simulink library "bat_13S7P_detailed"  (R2025b)
settings: Solver=VariableStepAuto  StartTime=0.0  StopTime=10.0  RelTol=1e-3
undefined symbols (not defined in the file or in its folder): battery_builder_rtmsupport, gcbh
libraries: bat_13S7P_detailed_lib x14
settings Model: Creator=scb4  LastModifiedBy=scb4

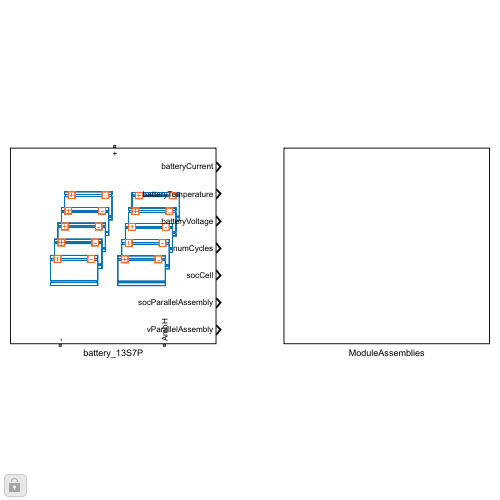
[thumbnail: Simulink's stored preview of the top-level diagram]
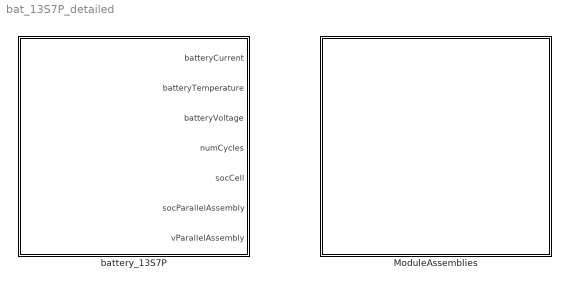
== system bat_13S7P_detailed ==
  ModuleAssemblies : Subsystem
  battery_13S7P : Subsystem  LoadFcn=battery_builder_rtmsupport('loadfcn',gcbh);
      settings: CopyFcn=battery_builder_rtmsupport('copyfcn',gcbh);  PreCopyFcn=battery_builder_rtmsupport('precopyfcn',gcbh);  PreDeleteFcn=battery_builder_rtmsupport('predeletefcn',gcbh);  PortSchema="{\"entries\":[{\"content\":{\"sides\":[{\"content\":{\"connectorIds\":[\"LConn1\"]},\"type\":\"ConnectorPlacement.EquallySpacedRectSide\",\"uuid\":\"c922c71b-bb80-4818-bdc8-e90d40dfbbb3\"},{\"content\":{\"connectorIds\":[\"RConn1\",\"RConn2\"],\"side\":\"RIGHT\"},\"type\":\"ConnectorPlacement.EquallySpacedRectSide\",\"uuid\":\"8cfcb0b4-3cbc-4068-a33f-0ddf2418c87b\"},{\"content\":{\"side\":\"TOP\"},\"type\":\"ConnectorPlacement.EquallySpacedRectSide\",\"uuid\":\"a3bda4bf-8d06-4bf0-ab5f-e835ee1e9452\"},{\"content\":{\"connectorIds\":[\"Out1\",\"Out2\",\"Out3\",\"Out4\",\"Out5\",\"Out6\",\"Out7\"],\"side\":\"BOTTOM\"},\"type\":\"ConnectorPlacement.EquallySpacedRectSide\",\"uuid\":\"4dc4e40d-eeb2-4e6c-ad84-aff3d30c3561\"}]},\"type\":\"ConnectorPlacement.EquallySpacedConnector\",\"uuid\":\"9bf5a596-b0f6-40a9-8ffe-ca0735a12662\"}],\"packageUris\":[\"http://schema.mathworks.com/mf0/Connector/R2020b\"],\"version\":\"1.0\"}"
      mask Display: image('$imagefile')

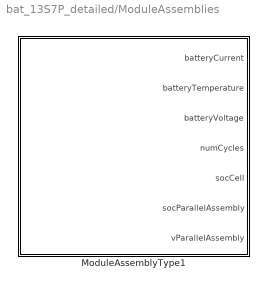
== system bat_13S7P_detailed/ModuleAssemblies ==
  ModuleAssemblyType1 : Subsystem  LoadFcn=battery_builder_rtmsupport('loadfcn',gcbh);
      settings: CopyFcn=battery_builder_rtmsupport('copyfcn',gcbh);  PreCopyFcn=battery_builder_rtmsupport('precopyfcn',gcbh);  PreDeleteFcn=battery_builder_rtmsupport('predeletefcn',gcbh);  PortSchema="{\"entries\":[{\"content\":{\"sides\":[{\"content\":{\"connectorIds\":[\"LConn1\"]},\"type\":\"ConnectorPlacement.EquallySpacedRectSide\",\"uuid\":\"c922c71b-bb80-4818-bdc8-e90d40dfbbb3\"},{\"content\":{\"connectorIds\":[\"RConn1\",\"RConn2\"],\"side\":\"RIGHT\"},\"type\":\"ConnectorPlacement.EquallySpacedRectSide\",\"uuid\":\"8cfcb0b4-3cbc-4068-a33f-0ddf2418c87b\"},{\"content\":{\"side\":\"TOP\"},\"type\":\"ConnectorPlacement.EquallySpacedRectSide\",\"uuid\":\"a3bda4bf-8d06-4bf0-ab5f-e835ee1e9452\"},{\"content\":{\"connectorIds\":[\"Out1\",\"Out2\",\"Out3\",\"Out4\",\"Out5\",\"Out6\",\"Out7\"],\"side\":\"BOTTOM\"},\"type\":\"ConnectorPlacement.EquallySpacedRectSide\",\"uuid\":\"a7aca7be-b7c9-453c-ab2d-6778c2fb4d01\"}]},\"type\":\"ConnectorPlacement.EquallySpacedConnector\",\"uuid\":\"9bf5a596-b0f6-40a9-8ffe-ca0735a12662\"}],\"packageUris\":[\"http://schema.mathworks.com/mf0/Connector/R2020b\"],\"version\":\"1.0\"}"
      mask Display: image('$imagefile')

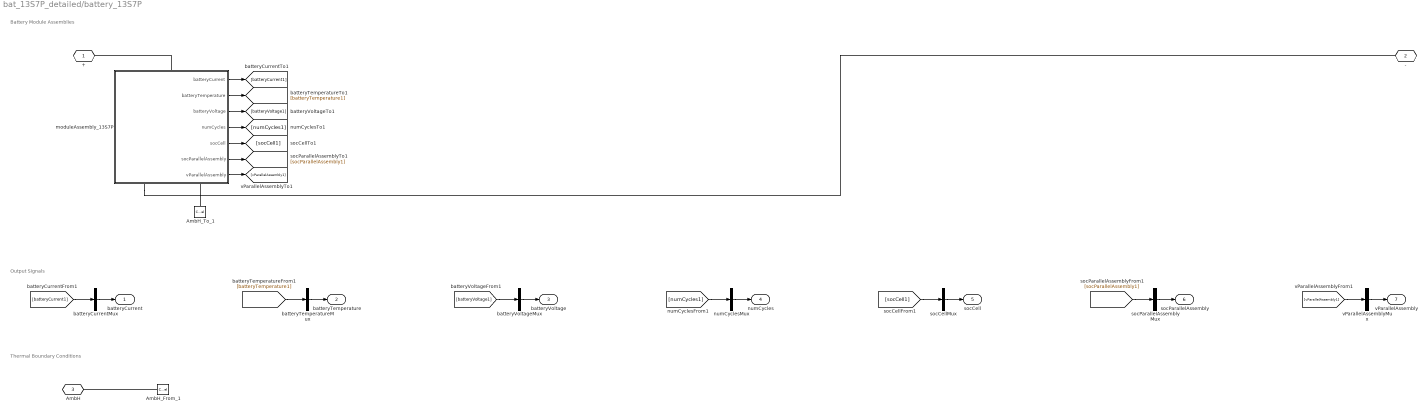
== system bat_13S7P_detailed/battery_13S7P ==
  note: Battery Module Assemblies
  note: Output Signals
  note: Thermal Boundary Conditions
  AmbH_From_1 : ConnectionLabel  Label=ambH_1
  AmbH_To_1 : ConnectionLabel  Label=ambH_1
  batteryCurrentMux : Mux  Inputs=1
  batteryTemperatureMux : Mux  Inputs=1
  batteryVoltageMux : Mux  Inputs=1
  moduleAssembly_13S7P : Subsystem  LoadFcn=battery_builder_rtmsupport('loadfcn',gcbh);
      settings: CopyFcn=battery_builder_rtmsupport('copyfcn',gcbh);  PreCopyFcn=battery_builder_rtmsupport('precopyfcn',gcbh);  PreDeleteFcn=battery_builder_rtmsupport('predeletefcn',gcbh);  PortSchema="{\"entries\":[{\"content\":{\"sides\":[{\"content\":{\"connectorIds\":[\"LConn1\"]},\"type\":\"ConnectorPlacement.EquallySpacedRectSide\",\"uuid\":\"c922c71b-bb80-4818-bdc8-e90d40dfbbb3\"},{\"content\":{\"connectorIds\":[\"RConn1\",\"RConn2\"],\"side\":\"RIGHT\"},\"type\":\"ConnectorPlacement.EquallySpacedRectSide\",\"uuid\":\"8cfcb0b4-3cbc-4068-a33f-0ddf2418c87b\"},{\"content\":{\"side\":\"TOP\"},\"type\":\"ConnectorPlacement.EquallySpacedRectSide\",\"uuid\":\"a3bda4bf-8d06-4bf0-ab5f-e835ee1e9452\"},{\"content\":{\"connectorIds\":[\"Out1\",\"Out2\",\"Out3\",\"Out4\",\"Out5\",\"Out6\",\"Out7\"],\"side\":\"BOTTOM\"},\"type\":\"ConnectorPlacement.EquallySpacedRectSide\",\"uuid\":\"a7aca7be-b7c9-453c-ab2d-6778c2fb4d01\"}]},\"type\":\"ConnectorPlacement.EquallySpacedConnector\",\"uuid\":\"9bf5a596-b0f6-40a9-8ffe-ca0735a12662\"}],\"packageUris\":[\"http://schema.mathworks.com/mf0/Connector/R2020b\"],\"version\":\"1.0\"}"
      mask Display: image('$imagefile')
  numCyclesMux : Mux  Inputs=1
  socCellMux : Mux  Inputs=1
  socParallelAssemblyMux : Mux  Inputs=1
  vParallelAssemblyMux : Mux  Inputs=1
  + : PMIOPort  Side=Left
  - : PMIOPort  Port=2  Side=Right
  AmbH : PMIOPort  Port=3  Side=Right  ConnectionType=Connection: foundation.thermal.thermal
  batteryCurrent : Outport
  batteryTemperature : Outport  Port=2
  batteryVoltage : Outport  Port=3
  numCycles : Outport  Port=4
  socCell : Outport  Port=5
  socParallelAssembly : Outport  Port=6
  vParallelAssembly : Outport  Port=7
  wires:
  moduleAssembly_13S7P/1(batteryCurrent) -> [batteryCurrent1]
  batteryCurrentMux/1 -> batteryCurrent/1
  [batteryCurrent1] -> batteryCurrentMux/1
  moduleAssembly_13S7P/2(batteryTemperature) -> [batteryTemperature1]
  batteryTemperatureMux/1 -> batteryTemperature/1
  [batteryTemperature1] -> batteryTemperatureMux/1
  moduleAssembly_13S7P/3(batteryVoltage) -> [batteryVoltage1]
  batteryVoltageMux/1 -> batteryVoltage/1
  [batteryVoltage1] -> batteryVoltageMux/1
  moduleAssembly_13S7P/4(numCycles) -> [numCycles1]
  numCyclesMux/1 -> numCycles/1
  [numCycles1] -> numCyclesMux/1
  moduleAssembly_13S7P/5(socCell) -> [socCell1]
  socCellMux/1 -> socCell/1
  [socCell1] -> socCellMux/1
  moduleAssembly_13S7P/6(socParallelAssembly) -> [socParallelAssembly1]
  socParallelAssemblyMux/1 -> socParallelAssembly/1
  [socParallelAssembly1] -> socParallelAssemblyMux/1
  moduleAssembly_13S7P/7(vParallelAssembly) -> [vParallelAssembly1]
  vParallelAssemblyMux/1 -> vParallelAssembly/1
  [vParallelAssembly1] -> vParallelAssemblyMux/1
  connections:
  moduleAssembly_13S7P/LConn1 -- +/RConn1
  moduleAssembly_13S7P/RConn1 -- -/RConn1
  AmbH_To_1/LConn1 -- moduleAssembly_13S7P/RConn2
  AmbH_From_1/LConn1 -- AmbH/RConn1

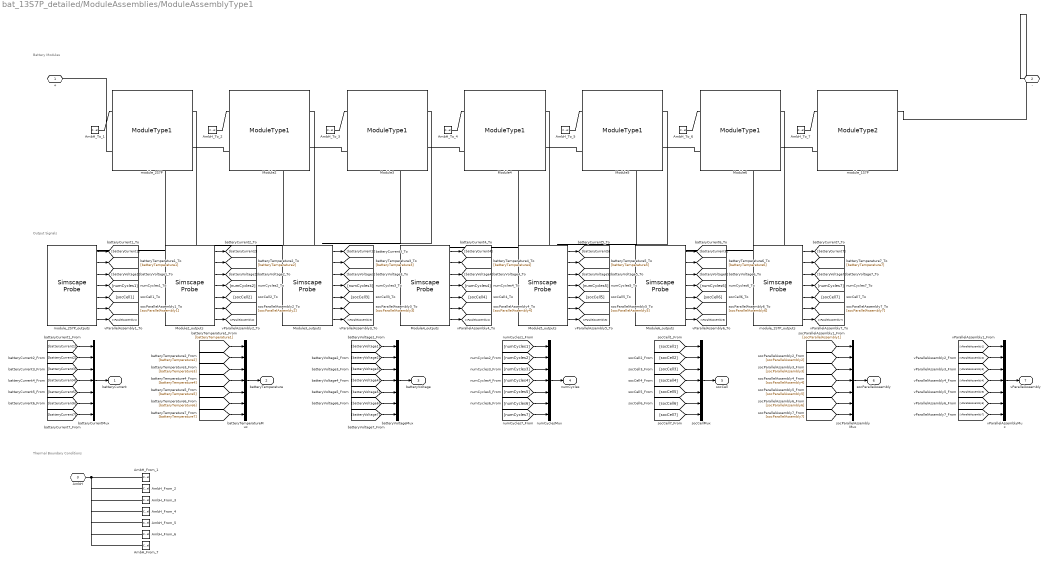
== system bat_13S7P_detailed/ModuleAssemblies/ModuleAssemblyType1 ==
  note: Battery Modules
  note: Output Signals
  note: Thermal Boundary Conditions
  AmbH_From_1 : ConnectionLabel  Label=ambH_1
  AmbH_From_2 : ConnectionLabel  Label=ambH_2
  AmbH_From_3 : ConnectionLabel  Label=ambH_3
  AmbH_From_4 : ConnectionLabel  Label=ambH_4
  AmbH_From_5 : ConnectionLabel  Label=ambH_5
  AmbH_From_6 : ConnectionLabel  Label=ambH_6
  AmbH_From_7 : ConnectionLabel  Label=ambH_7
  AmbH_To_1 : ConnectionLabel  Label=ambH_1
  AmbH_To_2 : ConnectionLabel  Label=ambH_2
  AmbH_To_3 : ConnectionLabel  Label=ambH_3
  AmbH_To_4 : ConnectionLabel  Label=ambH_4
  AmbH_To_5 : ConnectionLabel  Label=ambH_5
  AmbH_To_6 : ConnectionLabel  Label=ambH_6
  AmbH_To_7 : ConnectionLabel  Label=ambH_7
  Module{2..6} (5 alike) : bat_13S7P_detailed_lib/Modules/ModuleType1  BatteryCapacityCell=ModuleType1.BatteryCapacityCell A*hr  ExtrapolationMethodCell=simscape.enum.extrapolation.nearest  SOCBreakpointsCell=ModuleType1.SOCBreakpointsCell  TemperatureBreakpointsCell=ModuleType1.TemperatureBreakpointsCell K  OpenCircuitVoltageThermalCell=ModuleType1.OpenCircuitVoltageThermalCell V  VoltageRangeCell=ModuleType1.VoltageRangeCell V  ResistanceSOCBreakpointsCell=ModuleType1.ResistanceSOCBreakpointsCell  ResistanceTemperatureBreakpointsCell=ModuleType1.ResistanceTemperatureBreakpointsCell K  R0ThermalCell=ModuleType1.R0ThermalCell Ohm  R1ThermalCell=ModuleType1.R1ThermalCell Ohm  Tau1ThermalCell=ModuleType1.Tau1ThermalCell s  BatteryThermalMassCell=ModuleType1.BatteryThermalMassCell J/K  AmbientResistance=ModuleType1.AmbientResistance K/W  P=7  S=2  socCell_specify=off  socCell_priority=High  socCell=repmat(1, 14, 1)  socCell_nominal_specify=off  socCell_nominal_value=1  socCell_nominal_unit=1  batteryVoltage_specify=off  batteryVoltage_priority=None  batteryVoltage=repmat(0, 14, 1) V  batteryVoltage_nominal_specify=off  batteryVoltage_nominal_value=1  batteryVoltage_nominal_unit=V  batteryCurrent_specify=off  batteryCurrent_priority=None  batteryCurrent=repmat(0, 14, 1) A  batteryCurrent_nominal_specify=off  batteryCurrent_nominal_value=1  batteryCurrent_nominal_unit=A  numCycles_specify=off  numCycles_priority=High  numCycles=repmat(0, 14, 1)  numCycles_nominal_specify=off  numCycles_nominal_value=1  numCycles_nominal_unit=1  batteryTemperature_specify=off  batteryTemperature_priority=High  batteryTemperature=repmat(298.15, 14, 1) K  batteryTemperature_nominal_specify=off  batteryTemperature_nominal_value=1  batteryTemperature_nominal_unit=K  vParallelAssembly_specify=off  vParallelAssembly_priority=None  vParallelAssembly=repmat(0, 2, 1) V  vParallelAssembly_nominal_specify=off  vParallelAssembly_nominal_value=1  vParallelAssembly_nominal_unit=V  socParallelAssembly_specify=off  socParallelAssembly_priority=None  socParallelAssembly=repmat(1, 2, 1)  socParallelAssembly_nominal_specify=off  socParallelAssembly_nominal_value=1  socParallelAssembly_nominal_unit=1
      settings: InternalSimscapePortConfiguration="{\"Bottom\":[{\"id\":\"n\",\"label\":\"-\",\"type\":\"foundation.electrical.electrical\"},{\"id\":\"BottomExtClnt\",\"label\":\"CPB\",\"type\":\"foundation.thermal.thermal\"}],\"Left\":[{\"id\":\"AmbH\",\"label\":\"AmbH\",\"type\":\"foundation.thermal.thermal\"}],\"Right\":[],\"Top\":[{\"id\":\"p\",\"label\":\"+\",\"type\":\"foundation.electrical.electrical\"}]}"
  Module2_outputs : SimscapeProbe  BoundBlock=4  Variables="{\"batteryCurrent\":{\"Probing\":\"ON\"},\"batteryTemperature\":{\"Probing\":\"ON\"},\"batteryVoltage\":{\"Probing\":\"ON\"},\"numCycles\":{\"Probing\":\"ON\"},\"socCell\":{\"Probing\":\"ON\"},\"socParallelAssembly\":{\"Probing\":\"ON\"},\"vParallelAssembly\":{\"Probing\":\"ON\"}}"
  Module3_outputs : SimscapeProbe  BoundBlock=5  Variables="{\"batteryCurrent\":{\"Probing\":\"ON\"},\"batteryTemperature\":{\"Probing\":\"ON\"},\"batteryVoltage\":{\"Probing\":\"ON\"},\"numCycles\":{\"Probing\":\"ON\"},\"socCell\":{\"Probing\":\"ON\"},\"socParallelAssembly\":{\"Probing\":\"ON\"},\"vParallelAssembly\":{\"Probing\":\"ON\"}}"
  Module4_outputs : SimscapeProbe  BoundBlock=6  Variables="{\"batteryCurrent\":{\"Probing\":\"ON\"},\"batteryTemperature\":{\"Probing\":\"ON\"},\"batteryVoltage\":{\"Probing\":\"ON\"},\"numCycles\":{\"Probing\":\"ON\"},\"socCell\":{\"Probing\":\"ON\"},\"socParallelAssembly\":{\"Probing\":\"ON\"},\"vParallelAssembly\":{\"Probing\":\"ON\"}}"
  Module5_outputs : SimscapeProbe  BoundBlock=7  Variables="{\"batteryCurrent\":{\"Probing\":\"ON\"},\"batteryTemperature\":{\"Probing\":\"ON\"},\"batteryVoltage\":{\"Probing\":\"ON\"},\"numCycles\":{\"Probing\":\"ON\"},\"socCell\":{\"Probing\":\"ON\"},\"socParallelAssembly\":{\"Probing\":\"ON\"},\"vParallelAssembly\":{\"Probing\":\"ON\"}}"
  Module6_outputs : SimscapeProbe  BoundBlock=8  Variables="{\"batteryCurrent\":{\"Probing\":\"ON\"},\"batteryTemperature\":{\"Probing\":\"ON\"},\"batteryVoltage\":{\"Probing\":\"ON\"},\"numCycles\":{\"Probing\":\"ON\"},\"socCell\":{\"Probing\":\"ON\"},\"socParallelAssembly\":{\"Probing\":\"ON\"},\"vParallelAssembly\":{\"Probing\":\"ON\"}}"
  batteryCurrentMux : Mux  Inputs=7
  batteryTemperatureMux : Mux  Inputs=7
  batteryVoltageMux : Mux  Inputs=7
  module_1S7P : bat_13S7P_detailed_lib/Modules/ModuleType2  BatteryCapacityCell=ModuleType2.BatteryCapacityCell A*hr  ExtrapolationMethodCell=simscape.enum.extrapolation.nearest  SOCBreakpointsCell=ModuleType2.SOCBreakpointsCell  TemperatureBreakpointsCell=ModuleType2.TemperatureBreakpointsCell K  OpenCircuitVoltageThermalCell=ModuleType2.OpenCircuitVoltageThermalCell V  VoltageRangeCell=ModuleType2.VoltageRangeCell V  ResistanceSOCBreakpointsCell=ModuleType2.ResistanceSOCBreakpointsCell  ResistanceTemperatureBreakpointsCell=ModuleType2.ResistanceTemperatureBreakpointsCell K  R0ThermalCell=ModuleType2.R0ThermalCell Ohm  R1ThermalCell=ModuleType2.R1ThermalCell Ohm  Tau1ThermalCell=ModuleType2.Tau1ThermalCell s  BatteryThermalMassCell=ModuleType2.BatteryThermalMassCell J/K  AmbientResistance=ModuleType2.AmbientResistance K/W  P=7  S=1  socCell_specify=off  socCell_priority=High  socCell=repmat(1, 7, 1)  socCell_nominal_specify=off  socCell_nominal_value=1  socCell_nominal_unit=1  batteryVoltage_specify=off  batteryVoltage_priority=None  batteryVoltage=repmat(0, 7, 1) V  batteryVoltage_nominal_specify=off  batteryVoltage_nominal_value=1  batteryVoltage_nominal_unit=V  batteryCurrent_specify=off  batteryCurrent_priority=None  batteryCurrent=repmat(0, 7, 1) A  batteryCurrent_nominal_specify=off  batteryCurrent_nominal_value=1  batteryCurrent_nominal_unit=A  numCycles_specify=off  numCycles_priority=High  numCycles=repmat(0, 7, 1)  numCycles_nominal_specify=off  numCycles_nominal_value=1  numCycles_nominal_unit=1  batteryTemperature_specify=off  batteryTemperature_priority=High  batteryTemperature=repmat(298.15, 7, 1) K  batteryTemperature_nominal_specify=off  batteryTemperature_nominal_value=1  batteryTemperature_nominal_unit=K  vParallelAssembly_specify=off  vParallelAssembly_priority=None  vParallelAssembly=0 V  vParallelAssembly_nominal_specify=off  vParallelAssembly_nominal_value=1  vParallelAssembly_nominal_unit=V  socParallelAssembly_specify=off  socParallelAssembly_priority=None  socParallelAssembly=1  socParallelAssembly_nominal_specify=off  socParallelAssembly_nominal_value=1  socParallelAssembly_nominal_unit=1
      settings: InternalSimscapePortConfiguration="{\"Bottom\":[{\"id\":\"n\",\"label\":\"-\",\"type\":\"foundation.electrical.electrical\"},{\"id\":\"BottomExtClnt\",\"label\":\"CPB\",\"type\":\"foundation.thermal.thermal\"}],\"Left\":[{\"id\":\"AmbH\",\"label\":\"AmbH\",\"type\":\"foundation.thermal.thermal\"}],\"Right\":[],\"Top\":[{\"id\":\"p\",\"label\":\"+\",\"type\":\"foundation.electrical.electrical\"}]}"
  module_1S7P_outputs : SimscapeProbe  BoundBlock=9  Variables="{\"batteryCurrent\":{\"Probing\":\"ON\"},\"batteryTemperature\":{\"Probing\":\"ON\"},\"batteryVoltage\":{\"Probing\":\"ON\"},\"numCycles\":{\"Probing\":\"ON\"},\"socCell\":{\"Probing\":\"ON\"},\"socParallelAssembly\":{\"Probing\":\"ON\"},\"vParallelAssembly\":{\"Probing\":\"ON\"}}"
  module_2S7P : bat_13S7P_detailed_lib/Modules/ModuleType1  BatteryCapacityCell=ModuleType1.BatteryCapacityCell A*hr  ExtrapolationMethodCell=simscape.enum.extrapolation.nearest  SOCBreakpointsCell=ModuleType1.SOCBreakpointsCell  TemperatureBreakpointsCell=ModuleType1.TemperatureBreakpointsCell K  OpenCircuitVoltageThermalCell=ModuleType1.OpenCircuitVoltageThermalCell V  VoltageRangeCell=ModuleType1.VoltageRangeCell V  ResistanceSOCBreakpointsCell=ModuleType1.ResistanceSOCBreakpointsCell  ResistanceTemperatureBreakpointsCell=ModuleType1.ResistanceTemperatureBreakpointsCell K  R0ThermalCell=ModuleType1.R0ThermalCell Ohm  R1ThermalCell=ModuleType1.R1ThermalCell Ohm  Tau1ThermalCell=ModuleType1.Tau1ThermalCell s  BatteryThermalMassCell=ModuleType1.BatteryThermalMassCell J/K  AmbientResistance=ModuleType1.AmbientResistance K/W  P=7  S=2  socCell_specify=off  socCell_priority=High  socCell=repmat(1, 14, 1)  socCell_nominal_specify=off  socCell_nominal_value=1  socCell_nominal_unit=1  batteryVoltage_specify=off  batteryVoltage_priority=None  batteryVoltage=repmat(0, 14, 1) V  batteryVoltage_nominal_specify=off  batteryVoltage_nominal_value=1  batteryVoltage_nominal_unit=V  batteryCurrent_specify=off  batteryCurrent_priority=None  batteryCurrent=repmat(0, 14, 1) A  batteryCurrent_nominal_specify=off  batteryCurrent_nominal_value=1  batteryCurrent_nominal_unit=A  numCycles_specify=off  numCycles_priority=High  numCycles=repmat(0, 14, 1)  numCycles_nominal_specify=off  numCycles_nominal_value=1  numCycles_nominal_unit=1  batteryTemperature_specify=off  batteryTemperature_priority=High  batteryTemperature=repmat(298.15, 14, 1) K  batteryTemperature_nominal_specify=off  batteryTemperature_nominal_value=1  batteryTemperature_nominal_unit=K  vParallelAssembly_specify=off  vParallelAssembly_priority=None  vParallelAssembly=repmat(0, 2, 1) V  vParallelAssembly_nominal_specify=off  vParallelAssembly_nominal_value=1  vParallelAssembly_nominal_unit=V  socParallelAssembly_specify=off  socParallelAssembly_priority=None  socParallelAssembly=repmat(1, 2, 1)  socParallelAssembly_nominal_specify=off  socParallelAssembly_nominal_value=1  socParallelAssembly_nominal_unit=1
      settings: InternalSimscapePortConfiguration="{\"Bottom\":[{\"id\":\"n\",\"label\":\"-\",\"type\":\"foundation.electrical.electrical\"},{\"id\":\"BottomExtClnt\",\"label\":\"CPB\",\"type\":\"foundation.thermal.thermal\"}],\"Left\":[{\"id\":\"AmbH\",\"label\":\"AmbH\",\"type\":\"foundation.thermal.thermal\"}],\"Right\":[],\"Top\":[{\"id\":\"p\",\"label\":\"+\",\"type\":\"foundation.electrical.electrical\"}]}"
  module_2S7P_outputs : SimscapeProbe  BoundBlock=3  Variables="{\"batteryCurrent\":{\"Probing\":\"ON\"},\"batteryTemperature\":{\"Probing\":\"ON\"},\"batteryVoltage\":{\"Probing\":\"ON\"},\"numCycles\":{\"Probing\":\"ON\"},\"socCell\":{\"Probing\":\"ON\"},\"socParallelAssembly\":{\"Probing\":\"ON\"},\"vParallelAssembly\":{\"Probing\":\"ON\"}}"
  numCyclesMux : Mux  Inputs=7
  socCellMux : Mux  Inputs=7
  socParallelAssemblyMux : Mux  Inputs=7
  vParallelAssemblyMux : Mux  Inputs=7
  + : PMIOPort  Side=Left
  - : PMIOPort  Port=2  Side=Right
  AmbH : PMIOPort  Port=3  Side=Right  ConnectionType=Connection: foundation.thermal.thermal
  batteryCurrent : Outport
  batteryTemperature : Outport  Port=2
  batteryVoltage : Outport  Port=3
  numCycles : Outport  Port=4
  socCell : Outport  Port=5
  socParallelAssembly : Outport  Port=6
  vParallelAssembly : Outport  Port=7
  wires:
  module_2S7P_outputs/1 -> [batteryCurrent1]
  batteryCurrentMux/1 -> batteryCurrent/1
  [batteryCurrent1] -> batteryCurrentMux/1
  module_2S7P_outputs/2 -> [batteryTemperature1]
  batteryTemperatureMux/1 -> batteryTemperature/1
  [batteryTemperature1] -> batteryTemperatureMux/1
  module_2S7P_outputs/3 -> [batteryVoltage1]
  batteryVoltageMux/1 -> batteryVoltage/1
  [batteryVoltage1] -> batteryVoltageMux/1
  module_2S7P_outputs/4 -> [numCycles1]
  numCyclesMux/1 -> numCycles/1
  [numCycles1] -> numCyclesMux/1
  module_2S7P_outputs/5 -> [socCell1]
  socCellMux/1 -> socCell/1
  [socCell1] -> socCellMux/1
  module_2S7P_outputs/6 -> [socParallelAssembly1]
  socParallelAssemblyMux/1 -> socParallelAssembly/1
  [socParallelAssembly1] -> socParallelAssemblyMux/1
  module_2S7P_outputs/7 -> [vParallelAssembly1]
  vParallelAssemblyMux/1 -> vParallelAssembly/1
  [vParallelAssembly1] -> vParallelAssemblyMux/1
  Module2_outputs/1 -> [batteryCurrent2]
  [batteryCurrent2] -> batteryCurrentMux/2
  Module2_outputs/2 -> [batteryTemperature2]
  [batteryTemperature2] -> batteryTemperatureMux/2
  Module2_outputs/3 -> [batteryVoltage2]
  [batteryVoltage2] -> batteryVoltageMux/2
  Module2_outputs/4 -> [numCycles2]
  [numCycles2] -> numCyclesMux/2
  Module2_outputs/5 -> [socCell2]
  [socCell2] -> socCellMux/2
  Module2_outputs/6 -> [socParallelAssembly2]
  [socParallelAssembly2] -> socParallelAssemblyMux/2
  Module2_outputs/7 -> [vParallelAssembly2]
  [vParallelAssembly2] -> vParallelAssemblyMux/2
  Module3_outputs/1 -> [batteryCurrent3]
  [batteryCurrent3] -> batteryCurrentMux/3
  Module3_outputs/2 -> [batteryTemperature3]
  [batteryTemperature3] -> batteryTemperatureMux/3
  Module3_outputs/3 -> [batteryVoltage3]
  [batteryVoltage3] -> batteryVoltageMux/3
  Module3_outputs/4 -> [numCycles3]
  [numCycles3] -> numCyclesMux/3
  Module3_outputs/5 -> [socCell3]
  [socCell3] -> socCellMux/3
  Module3_outputs/6 -> [socParallelAssembly3]
  [socParallelAssembly3] -> socParallelAssemblyMux/3
  Module3_outputs/7 -> [vParallelAssembly3]
  [vParallelAssembly3] -> vParallelAssemblyMux/3
  Module4_outputs/1 -> [batteryCurrent4]
  [batteryCurrent4] -> batteryCurrentMux/4
  Module4_outputs/2 -> [batteryTemperature4]
  [batteryTemperature4] -> batteryTemperatureMux/4
  Module4_outputs/3 -> [batteryVoltage4]
  [batteryVoltage4] -> batteryVoltageMux/4
  Module4_outputs/4 -> [numCycles4]
  [numCycles4] -> numCyclesMux/4
  Module4_outputs/5 -> [socCell4]
  [socCell4] -> socCellMux/4
  Module4_outputs/6 -> [socParallelAssembly4]
  [socParallelAssembly4] -> socParallelAssemblyMux/4
  Module4_outputs/7 -> [vParallelAssembly4]
  [vParallelAssembly4] -> vParallelAssemblyMux/4
  Module5_outputs/1 -> [batteryCurrent5]
  [batteryCurrent5] -> batteryCurrentMux/5
  Module5_outputs/2 -> [batteryTemperature5]
  [batteryTemperature5] -> batteryTemperatureMux/5
  Module5_outputs/3 -> [batteryVoltage5]
  [batteryVoltage5] -> batteryVoltageMux/5
  Module5_outputs/4 -> [numCycles5]
  [numCycles5] -> numCyclesMux/5
  Module5_outputs/5 -> [socCell5]
  [socCell5] -> socCellMux/5
  Module5_outputs/6 -> [socParallelAssembly5]
  [socParallelAssembly5] -> socParallelAssemblyMux/5
  Module5_outputs/7 -> [vParallelAssembly5]
  [vParallelAssembly5] -> vParallelAssemblyMux/5
  Module6_outputs/1 -> [batteryCurrent6]
  [batteryCurrent6] -> batteryCurrentMux/6
  Module6_outputs/2 -> [batteryTemperature6]
  [batteryTemperature6] -> batteryTemperatureMux/6
  Module6_outputs/3 -> [batteryVoltage6]
  [batteryVoltage6] -> batteryVoltageMux/6
  Module6_outputs/4 -> [numCycles6]
  [numCycles6] -> numCyclesMux/6
  Module6_outputs/5 -> [socCell6]
  [socCell6] -> socCellMux/6
  Module6_outputs/6 -> [socParallelAssembly6]
  [socParallelAssembly6] -> socParallelAssemblyMux/6
  Module6_outputs/7 -> [vParallelAssembly6]
  [vParallelAssembly6] -> vParallelAssemblyMux/6
  module_1S7P_outputs/1 -> [batteryCurrent7]
  [batteryCurrent7] -> batteryCurrentMux/7
  module_1S7P_outputs/2 -> [batteryTemperature7]
  [batteryTemperature7] -> batteryTemperatureMux/7
  module_1S7P_outputs/3 -> [batteryVoltage7]
  [batteryVoltage7] -> batteryVoltageMux/7
  module_1S7P_outputs/4 -> [numCycles7]
  [numCycles7] -> numCyclesMux/7
  module_1S7P_outputs/5 -> [socCell7]
  [socCell7] -> socCellMux/7
  module_1S7P_outputs/6 -> [socParallelAssembly7]
  [socParallelAssembly7] -> socParallelAssemblyMux/7
  module_1S7P_outputs/7 -> [vParallelAssembly7]
  [vParallelAssembly7] -> vParallelAssemblyMux/7
  connections:
  Module2/LConn2 -- module_2S7P/RConn1
  Module3/LConn2 -- Module2/RConn1
  Module4/LConn2 -- Module3/RConn1
  Module5/LConn2 -- Module4/RConn1
  Module6/LConn2 -- Module5/RConn1
  module_1S7P/LConn2 -- Module6/RConn1
  module_2S7P/LConn2 -- +/RConn1
  module_1S7P/RConn1 -- -/RConn1
  AmbH_To_1/LConn1 -- module_2S7P/LConn1
  AmbH_From_1/LConn1 -- AmbH_From_2/LConn1 -- AmbH_From_3/LConn1 -- AmbH_From_4/LConn1 -- AmbH_From_5/LConn1 -- AmbH_From_6/LConn1 -- AmbH/RConn1 -- AmbH_From_7/LConn1
  AmbH_To_2/LConn1 -- Module2/LConn1
  AmbH_To_3/LConn1 -- Module3/LConn1
  AmbH_To_4/LConn1 -- Module4/LConn1
  AmbH_To_5/LConn1 -- Module5/LConn1
  AmbH_To_6/LConn1 -- Module6/LConn1
  AmbH_To_7/LConn1 -- module_1S7P/LConn1

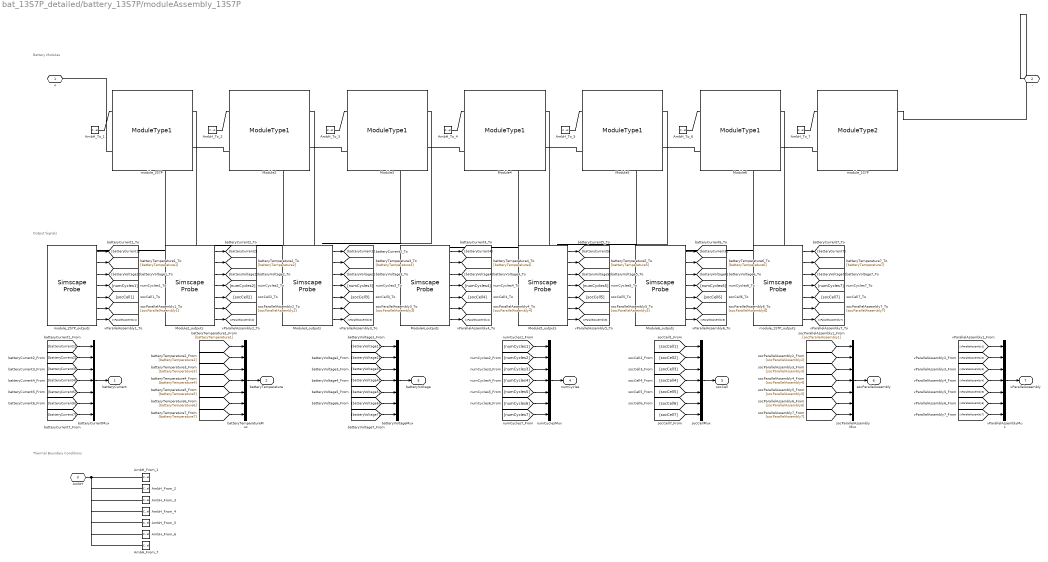
== system bat_13S7P_detailed/battery_13S7P/moduleAssembly_13S7P ==
  note: Thermal Boundary Conditions
  note: Output Signals
  note: Battery Modules
  AmbH_From_1 : ConnectionLabel  Label=ambH_1
  AmbH_From_2 : ConnectionLabel  Label=ambH_2
  AmbH_From_3 : ConnectionLabel  Label=ambH_3
  AmbH_From_4 : ConnectionLabel  Label=ambH_4
  AmbH_From_5 : ConnectionLabel  Label=ambH_5
  AmbH_From_6 : ConnectionLabel  Label=ambH_6
  AmbH_From_7 : ConnectionLabel  Label=ambH_7
  AmbH_To_1 : ConnectionLabel  Label=ambH_1
  AmbH_To_2 : ConnectionLabel  Label=ambH_2
  AmbH_To_3 : ConnectionLabel  Label=ambH_3
  AmbH_To_4 : ConnectionLabel  Label=ambH_4
  AmbH_To_5 : ConnectionLabel  Label=ambH_5
  AmbH_To_6 : ConnectionLabel  Label=ambH_6
  AmbH_To_7 : ConnectionLabel  Label=ambH_7
  Module{2..6} (5 alike) : bat_13S7P_detailed_lib/Modules/ModuleType1  BatteryCapacityCell=ModuleType1.BatteryCapacityCell A*hr  ExtrapolationMethodCell=simscape.enum.extrapolation.nearest  SOCBreakpointsCell=ModuleType1.SOCBreakpointsCell  TemperatureBreakpointsCell=ModuleType1.TemperatureBreakpointsCell K  OpenCircuitVoltageThermalCell=ModuleType1.OpenCircuitVoltageThermalCell V  VoltageRangeCell=ModuleType1.VoltageRangeCell V  ResistanceSOCBreakpointsCell=ModuleType1.ResistanceSOCBreakpointsCell  ResistanceTemperatureBreakpointsCell=ModuleType1.ResistanceTemperatureBreakpointsCell K  R0ThermalCell=ModuleType1.R0ThermalCell Ohm  R1ThermalCell=ModuleType1.R1ThermalCell Ohm  Tau1ThermalCell=ModuleType1.Tau1ThermalCell s  BatteryThermalMassCell=ModuleType1.BatteryThermalMassCell J/K  AmbientResistance=ModuleType1.AmbientResistance K/W  P=7  S=2  socCell_specify=off  socCell_priority=High  socCell=repmat(1, 14, 1)  socCell_nominal_specify=off  socCell_nominal_value=1  socCell_nominal_unit=1  batteryVoltage_specify=off  batteryVoltage_priority=None  batteryVoltage=repmat(0, 14, 1) V  batteryVoltage_nominal_specify=off  batteryVoltage_nominal_value=1  batteryVoltage_nominal_unit=V  batteryCurrent_specify=off  batteryCurrent_priority=None  batteryCurrent=repmat(0, 14, 1) A  batteryCurrent_nominal_specify=off  batteryCurrent_nominal_value=1  batteryCurrent_nominal_unit=A  numCycles_specify=off  numCycles_priority=High  numCycles=repmat(0, 14, 1)  numCycles_nominal_specify=off  numCycles_nominal_value=1  numCycles_nominal_unit=1  batteryTemperature_specify=off  batteryTemperature_priority=High  batteryTemperature=repmat(298.15, 14, 1) K  batteryTemperature_nominal_specify=off  batteryTemperature_nominal_value=1  batteryTemperature_nominal_unit=K  vParallelAssembly_specify=off  vParallelAssembly_priority=None  vParallelAssembly=repmat(0, 2, 1) V  vParallelAssembly_nominal_specify=off  vParallelAssembly_nominal_value=1  vParallelAssembly_nominal_unit=V  socParallelAssembly_specify=off  socParallelAssembly_priority=None  socParallelAssembly=repmat(1, 2, 1)  socParallelAssembly_nominal_specify=off  socParallelAssembly_nominal_value=1  socParallelAssembly_nominal_unit=1
      settings: InternalSimscapePortConfiguration="{\"Bottom\":[{\"id\":\"n\",\"label\":\"-\",\"type\":\"foundation.electrical.electrical\"},{\"id\":\"BottomExtClnt\",\"label\":\"CPB\",\"type\":\"foundation.thermal.thermal\"}],\"Left\":[{\"id\":\"AmbH\",\"label\":\"AmbH\",\"type\":\"foundation.thermal.thermal\"}],\"Right\":[],\"Top\":[{\"id\":\"p\",\"label\":\"+\",\"type\":\"foundation.electrical.electrical\"}]}"
  Module2_outputs : SimscapeProbe  BoundBlock=165  Variables="{\"batteryCurrent\":{\"Probing\":\"ON\"},\"batteryTemperature\":{\"Probing\":\"ON\"},\"batteryVoltage\":{\"Probing\":\"ON\"},\"numCycles\":{\"Probing\":\"ON\"},\"socCell\":{\"Probing\":\"ON\"},\"socParallelAssembly\":{\"Probing\":\"ON\"},\"vParallelAssembly\":{\"Probing\":\"ON\"}}"
  Module3_outputs : SimscapeProbe  BoundBlock=167  Variables="{\"batteryCurrent\":{\"Probing\":\"ON\"},\"batteryTemperature\":{\"Probing\":\"ON\"},\"batteryVoltage\":{\"Probing\":\"ON\"},\"numCycles\":{\"Probing\":\"ON\"},\"socCell\":{\"Probing\":\"ON\"},\"socParallelAssembly\":{\"Probing\":\"ON\"},\"vParallelAssembly\":{\"Probing\":\"ON\"}}"
  Module4_outputs : SimscapeProbe  BoundBlock=169  Variables="{\"batteryCurrent\":{\"Probing\":\"ON\"},\"batteryTemperature\":{\"Probing\":\"ON\"},\"batteryVoltage\":{\"Probing\":\"ON\"},\"numCycles\":{\"Probing\":\"ON\"},\"socCell\":{\"Probing\":\"ON\"},\"socParallelAssembly\":{\"Probing\":\"ON\"},\"vParallelAssembly\":{\"Probing\":\"ON\"}}"
  Module5_outputs : SimscapeProbe  BoundBlock=171  Variables="{\"batteryCurrent\":{\"Probing\":\"ON\"},\"batteryTemperature\":{\"Probing\":\"ON\"},\"batteryVoltage\":{\"Probing\":\"ON\"},\"numCycles\":{\"Probing\":\"ON\"},\"socCell\":{\"Probing\":\"ON\"},\"socParallelAssembly\":{\"Probing\":\"ON\"},\"vParallelAssembly\":{\"Probing\":\"ON\"}}"
  Module6_outputs : SimscapeProbe  BoundBlock=173  Variables="{\"batteryCurrent\":{\"Probing\":\"ON\"},\"batteryTemperature\":{\"Probing\":\"ON\"},\"batteryVoltage\":{\"Probing\":\"ON\"},\"numCycles\":{\"Probing\":\"ON\"},\"socCell\":{\"Probing\":\"ON\"},\"socParallelAssembly\":{\"Probing\":\"ON\"},\"vParallelAssembly\":{\"Probing\":\"ON\"}}"
  batteryCurrentMux : Mux  Inputs=7
  batteryTemperatureMux : Mux  Inputs=7
  batteryVoltageMux : Mux  Inputs=7
  module_1S7P : bat_13S7P_detailed_lib/Modules/ModuleType2  BatteryCapacityCell=ModuleType2.BatteryCapacityCell A*hr  ExtrapolationMethodCell=simscape.enum.extrapolation.nearest  SOCBreakpointsCell=ModuleType2.SOCBreakpointsCell  TemperatureBreakpointsCell=ModuleType2.TemperatureBreakpointsCell K  OpenCircuitVoltageThermalCell=ModuleType2.OpenCircuitVoltageThermalCell V  VoltageRangeCell=ModuleType2.VoltageRangeCell V  ResistanceSOCBreakpointsCell=ModuleType2.ResistanceSOCBreakpointsCell  ResistanceTemperatureBreakpointsCell=ModuleType2.ResistanceTemperatureBreakpointsCell K  R0ThermalCell=ModuleType2.R0ThermalCell Ohm  R1ThermalCell=ModuleType2.R1ThermalCell Ohm  Tau1ThermalCell=ModuleType2.Tau1ThermalCell s  BatteryThermalMassCell=ModuleType2.BatteryThermalMassCell J/K  AmbientResistance=ModuleType2.AmbientResistance K/W  P=7  S=1  socCell_specify=off  socCell_priority=High  socCell=repmat(1, 7, 1)  socCell_nominal_specify=off  socCell_nominal_value=1  socCell_nominal_unit=1  batteryVoltage_specify=off  batteryVoltage_priority=None  batteryVoltage=repmat(0, 7, 1) V  batteryVoltage_nominal_specify=off  batteryVoltage_nominal_value=1  batteryVoltage_nominal_unit=V  batteryCurrent_specify=off  batteryCurrent_priority=None  batteryCurrent=repmat(0, 7, 1) A  batteryCurrent_nominal_specify=off  batteryCurrent_nominal_value=1  batteryCurrent_nominal_unit=A  numCycles_specify=off  numCycles_priority=High  numCycles=repmat(0, 7, 1)  numCycles_nominal_specify=off  numCycles_nominal_value=1  numCycles_nominal_unit=1  batteryTemperature_specify=off  batteryTemperature_priority=High  batteryTemperature=repmat(298.15, 7, 1) K  batteryTemperature_nominal_specify=off  batteryTemperature_nominal_value=1  batteryTemperature_nominal_unit=K  vParallelAssembly_specify=off  vParallelAssembly_priority=None  vParallelAssembly=0 V  vParallelAssembly_nominal_specify=off  vParallelAssembly_nominal_value=1  vParallelAssembly_nominal_unit=V  socParallelAssembly_specify=off  socParallelAssembly_priority=None  socParallelAssembly=1  socParallelAssembly_nominal_specify=off  socParallelAssembly_nominal_value=1  socParallelAssembly_nominal_unit=1
      settings: InternalSimscapePortConfiguration="{\"Bottom\":[{\"id\":\"n\",\"label\":\"-\",\"type\":\"foundation.electrical.electrical\"},{\"id\":\"BottomExtClnt\",\"label\":\"CPB\",\"type\":\"foundation.thermal.thermal\"}],\"Left\":[{\"id\":\"AmbH\",\"label\":\"AmbH\",\"type\":\"foundation.thermal.thermal\"}],\"Right\":[],\"Top\":[{\"id\":\"p\",\"label\":\"+\",\"type\":\"foundation.electrical.electrical\"}]}"
  module_1S7P_outputs : SimscapeProbe  BoundBlock=220  Variables="{\"batteryCurrent\":{\"Probing\":\"ON\"},\"batteryTemperature\":{\"Probing\":\"ON\"},\"batteryVoltage\":{\"Probing\":\"ON\"},\"numCycles\":{\"Probing\":\"ON\"},\"socCell\":{\"Probing\":\"ON\"},\"socParallelAssembly\":{\"Probing\":\"ON\"},\"vParallelAssembly\":{\"Probing\":\"ON\"}}"
  module_2S7P : bat_13S7P_detailed_lib/Modules/ModuleType1  BatteryCapacityCell=ModuleType1.BatteryCapacityCell A*hr  ExtrapolationMethodCell=simscape.enum.extrapolation.nearest  SOCBreakpointsCell=ModuleType1.SOCBreakpointsCell  TemperatureBreakpointsCell=ModuleType1.TemperatureBreakpointsCell K  OpenCircuitVoltageThermalCell=ModuleType1.OpenCircuitVoltageThermalCell V  VoltageRangeCell=ModuleType1.VoltageRangeCell V  ResistanceSOCBreakpointsCell=ModuleType1.ResistanceSOCBreakpointsCell  ResistanceTemperatureBreakpointsCell=ModuleType1.ResistanceTemperatureBreakpointsCell K  R0ThermalCell=ModuleType1.R0ThermalCell Ohm  R1ThermalCell=ModuleType1.R1ThermalCell Ohm  Tau1ThermalCell=ModuleType1.Tau1ThermalCell s  BatteryThermalMassCell=ModuleType1.BatteryThermalMassCell J/K  AmbientResistance=ModuleType1.AmbientResistance K/W  P=7  S=2  socCell_specify=off  socCell_priority=High  socCell=repmat(1, 14, 1)  socCell_nominal_specify=off  socCell_nominal_value=1  socCell_nominal_unit=1  batteryVoltage_specify=off  batteryVoltage_priority=None  batteryVoltage=repmat(0, 14, 1) V  batteryVoltage_nominal_specify=off  batteryVoltage_nominal_value=1  batteryVoltage_nominal_unit=V  batteryCurrent_specify=off  batteryCurrent_priority=None  batteryCurrent=repmat(0, 14, 1) A  batteryCurrent_nominal_specify=off  batteryCurrent_nominal_value=1  batteryCurrent_nominal_unit=A  numCycles_specify=off  numCycles_priority=High  numCycles=repmat(0, 14, 1)  numCycles_nominal_specify=off  numCycles_nominal_value=1  numCycles_nominal_unit=1  batteryTemperature_specify=off  batteryTemperature_priority=High  batteryTemperature=repmat(298.15, 14, 1) K  batteryTemperature_nominal_specify=off  batteryTemperature_nominal_value=1  batteryTemperature_nominal_unit=K  vParallelAssembly_specify=off  vParallelAssembly_priority=None  vParallelAssembly=repmat(0, 2, 1) V  vParallelAssembly_nominal_specify=off  vParallelAssembly_nominal_value=1  vParallelAssembly_nominal_unit=V  socParallelAssembly_specify=off  socParallelAssembly_priority=None  socParallelAssembly=repmat(1, 2, 1)  socParallelAssembly_nominal_specify=off  socParallelAssembly_nominal_value=1  socParallelAssembly_nominal_unit=1
      settings: InternalSimscapePortConfiguration="{\"Bottom\":[{\"id\":\"n\",\"label\":\"-\",\"type\":\"foundation.electrical.electrical\"},{\"id\":\"BottomExtClnt\",\"label\":\"CPB\",\"type\":\"foundation.thermal.thermal\"}],\"Left\":[{\"id\":\"AmbH\",\"label\":\"AmbH\",\"type\":\"foundation.thermal.thermal\"}],\"Right\":[],\"Top\":[{\"id\":\"p\",\"label\":\"+\",\"type\":\"foundation.electrical.electrical\"}]}"
  module_2S7P_outputs : SimscapeProbe  BoundBlock=222  Variables="{\"batteryCurrent\":{\"Probing\":\"ON\"},\"batteryTemperature\":{\"Probing\":\"ON\"},\"batteryVoltage\":{\"Probing\":\"ON\"},\"numCycles\":{\"Probing\":\"ON\"},\"socCell\":{\"Probing\":\"ON\"},\"socParallelAssembly\":{\"Probing\":\"ON\"},\"vParallelAssembly\":{\"Probing\":\"ON\"}}"
  numCyclesMux : Mux  Inputs=7
  socCellMux : Mux  Inputs=7
  socParallelAssemblyMux : Mux  Inputs=7
  vParallelAssemblyMux : Mux  Inputs=7
  + : PMIOPort  Side=Left
  - : PMIOPort  Port=2  Side=Right
  AmbH : PMIOPort  Port=3  Side=Right  ConnectionType=Connection: foundation.thermal.thermal
  batteryCurrent : Outport
  batteryTemperature : Outport  Port=2
  batteryVoltage : Outport  Port=3
  numCycles : Outport  Port=4
  socCell : Outport  Port=5
  socParallelAssembly : Outport  Port=6
  vParallelAssembly : Outport  Port=7
  wires:
  [vParallelAssembly7] -> vParallelAssemblyMux/7
  module_1S7P_outputs/7 -> [vParallelAssembly7]
  [socParallelAssembly7] -> socParallelAssemblyMux/7
  module_1S7P_outputs/6 -> [socParallelAssembly7]
  [socCell7] -> socCellMux/7
  module_1S7P_outputs/5 -> [socCell7]
  [numCycles7] -> numCyclesMux/7
  module_1S7P_outputs/4 -> [numCycles7]
  [batteryVoltage7] -> batteryVoltageMux/7
  module_1S7P_outputs/3 -> [batteryVoltage7]
  [batteryTemperature7] -> batteryTemperatureMux/7
  module_1S7P_outputs/2 -> [batteryTemperature7]
  [batteryCurrent7] -> batteryCurrentMux/7
  module_1S7P_outputs/1 -> [batteryCurrent7]
  [vParallelAssembly6] -> vParallelAssemblyMux/6
  Module6_outputs/7 -> [vParallelAssembly6]
  [socParallelAssembly6] -> socParallelAssemblyMux/6
  Module6_outputs/6 -> [socParallelAssembly6]
  [socCell6] -> socCellMux/6
  Module6_outputs/5 -> [socCell6]
  [numCycles6] -> numCyclesMux/6
  Module6_outputs/4 -> [numCycles6]
  [batteryVoltage6] -> batteryVoltageMux/6
  Module6_outputs/3 -> [batteryVoltage6]
  [batteryTemperature6] -> batteryTemperatureMux/6
  Module6_outputs/2 -> [batteryTemperature6]
  [batteryCurrent6] -> batteryCurrentMux/6
  Module6_outputs/1 -> [batteryCurrent6]
  [vParallelAssembly5] -> vParallelAssemblyMux/5
  Module5_outputs/7 -> [vParallelAssembly5]
  [socParallelAssembly5] -> socParallelAssemblyMux/5
  Module5_outputs/6 -> [socParallelAssembly5]
  [socCell5] -> socCellMux/5
  Module5_outputs/5 -> [socCell5]
  [numCycles5] -> numCyclesMux/5
  Module5_outputs/4 -> [numCycles5]
  [batteryVoltage5] -> batteryVoltageMux/5
  Module5_outputs/3 -> [batteryVoltage5]
  [batteryTemperature5] -> batteryTemperatureMux/5
  Module5_outputs/2 -> [batteryTemperature5]
  [batteryCurrent5] -> batteryCurrentMux/5
  Module5_outputs/1 -> [batteryCurrent5]
  [vParallelAssembly4] -> vParallelAssemblyMux/4
  Module4_outputs/7 -> [vParallelAssembly4]
  [socParallelAssembly4] -> socParallelAssemblyMux/4
  Module4_outputs/6 -> [socParallelAssembly4]
  [socCell4] -> socCellMux/4
  Module4_outputs/5 -> [socCell4]
  [numCycles4] -> numCyclesMux/4
  Module4_outputs/4 -> [numCycles4]
  [batteryVoltage4] -> batteryVoltageMux/4
  Module4_outputs/3 -> [batteryVoltage4]
  [batteryTemperature4] -> batteryTemperatureMux/4
  Module4_outputs/2 -> [batteryTemperature4]
  [batteryCurrent4] -> batteryCurrentMux/4
  Module4_outputs/1 -> [batteryCurrent4]
  [vParallelAssembly3] -> vParallelAssemblyMux/3
  Module3_outputs/7 -> [vParallelAssembly3]
  [socParallelAssembly3] -> socParallelAssemblyMux/3
  Module3_outputs/6 -> [socParallelAssembly3]
  [socCell3] -> socCellMux/3
  Module3_outputs/5 -> [socCell3]
  [numCycles3] -> numCyclesMux/3
  Module3_outputs/4 -> [numCycles3]
  [batteryVoltage3] -> batteryVoltageMux/3
  Module3_outputs/3 -> [batteryVoltage3]
  [batteryTemperature3] -> batteryTemperatureMux/3
  Module3_outputs/2 -> [batteryTemperature3]
  [batteryCurrent3] -> batteryCurrentMux/3
  Module3_outputs/1 -> [batteryCurrent3]
  [vParallelAssembly2] -> vParallelAssemblyMux/2
  Module2_outputs/7 -> [vParallelAssembly2]
  [socParallelAssembly2] -> socParallelAssemblyMux/2
  Module2_outputs/6 -> [socParallelAssembly2]
  [socCell2] -> socCellMux/2
  Module2_outputs/5 -> [socCell2]
  [numCycles2] -> numCyclesMux/2
  Module2_outputs/4 -> [numCycles2]
  [batteryVoltage2] -> batteryVoltageMux/2
  Module2_outputs/3 -> [batteryVoltage2]
  [batteryTemperature2] -> batteryTemperatureMux/2
  Module2_outputs/2 -> [batteryTemperature2]
  [batteryCurrent2] -> batteryCurrentMux/2
  Module2_outputs/1 -> [batteryCurrent2]
  [vParallelAssembly1] -> vParallelAssemblyMux/1
  vParallelAssemblyMux/1 -> vParallelAssembly/1
  module_2S7P_outputs/7 -> [vParallelAssembly1]
  [socParallelAssembly1] -> socParallelAssemblyMux/1
  socParallelAssemblyMux/1 -> socParallelAssembly/1
  module_2S7P_outputs/6 -> [socParallelAssembly1]
  [socCell1] -> socCellMux/1
  socCellMux/1 -> socCell/1
  module_2S7P_outputs/5 -> [socCell1]
  [numCycles1] -> numCyclesMux/1
  numCyclesMux/1 -> numCycles/1
  module_2S7P_outputs/4 -> [numCycles1]
  [batteryVoltage1] -> batteryVoltageMux/1
  batteryVoltageMux/1 -> batteryVoltage/1
  module_2S7P_outputs/3 -> [batteryVoltage1]
  [batteryTemperature1] -> batteryTemperatureMux/1
  batteryTemperatureMux/1 -> batteryTemperature/1
  module_2S7P_outputs/2 -> [batteryTemperature1]
  [batteryCurrent1] -> batteryCurrentMux/1
  batteryCurrentMux/1 -> batteryCurrent/1
  module_2S7P_outputs/1 -> [batteryCurrent1]
  connections:
  AmbH_To_7/LConn1 -- module_1S7P/LConn1
  AmbH_To_6/LConn1 -- Module6/LConn1
  AmbH_To_5/LConn1 -- Module5/LConn1
  AmbH_To_4/LConn1 -- Module4/LConn1
  AmbH_To_3/LConn1 -- Module3/LConn1
  AmbH_To_2/LConn1 -- Module2/LConn1
  AmbH_From_7/LConn1 -- AmbH/RConn1 -- AmbH_From_6/LConn1 -- AmbH_From_5/LConn1 -- AmbH_From_4/LConn1 -- AmbH_From_3/LConn1 -- AmbH_From_2/LConn1 -- AmbH_From_1/LConn1
  AmbH_To_1/LConn1 -- module_2S7P/LConn1
  module_1S7P/RConn1 -- -/RConn1
  module_2S7P/LConn2 -- +/RConn1
  module_1S7P/LConn2 -- Module6/RConn1
  Module6/LConn2 -- Module5/RConn1
  Module5/LConn2 -- Module4/RConn1
  Module4/LConn2 -- Module3/RConn1
  Module3/LConn2 -- Module2/RConn1
  Module2/LConn2 -- module_2S7P/RConn1
